simulink model "sensor_MAG_model"  (R2025b)
settings: Solver=FixedStepDiscrete  StartTime=0.0  StopTime=20  FixedStep=0.001  RelTol=1e-3
undefined symbols (not defined in the file or in its folder): IMU_SAMPLE_RATE, MAG_RANGE, MAG_SAMPLE_RATE
settings Model: DataDictionary=SensorDict.sldd  Creator=89447  LastModifiedBy=89447
settings DataIOCC: ExternalInput=S  LoadExternalInput=on

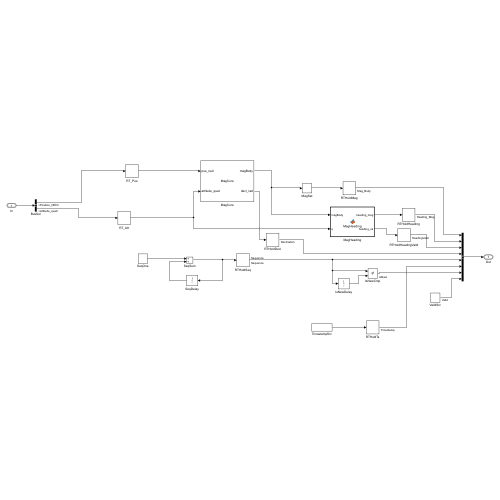
[thumbnail: Simulink's stored preview of the top-level diagram]
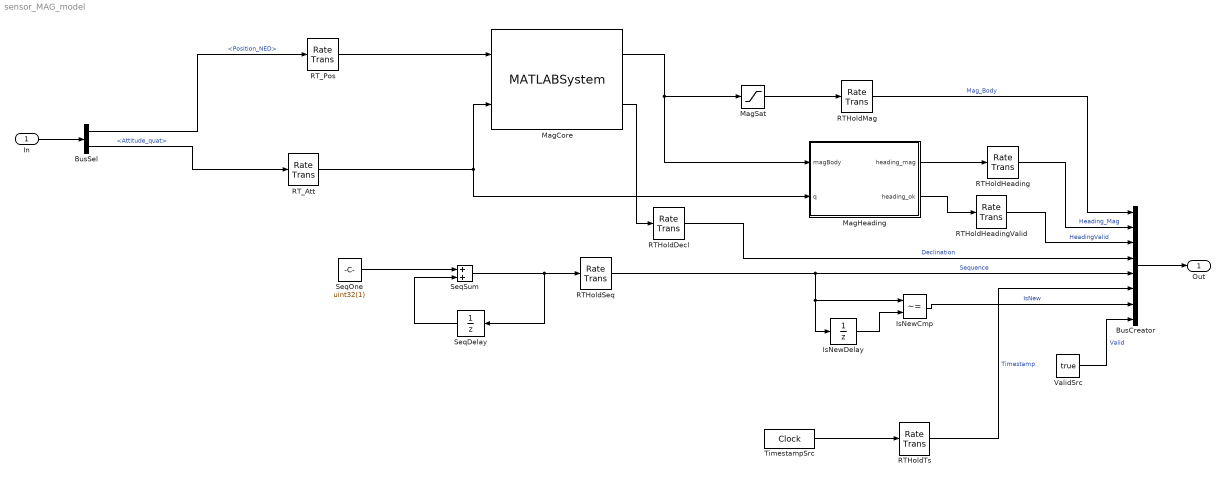
== system sensor_MAG_model ==
  In : Inport  OutDataTypeStr=Bus: DynamicModelBus
  BusCreator : BusCreator  Inputs=8  OutDataTypeStr=Bus: MagnetometerBus  NonVirtualBus=on
  BusSel : BusSelector  OutputSignals=Position_NED,Attitude_quat
  IsNewCmp : RelationalOperator  Operator=~=  OutDataTypeStr=boolean  RndMeth=Simplest  InputSameDT=off
  IsNewDelay : UnitDelay  SampleTime=1/double(IMU_SAMPLE_RATE)  HasFrameUpgradeWarning=on
  MagCore : MATLABSystem  System=MagCore  SampleRate=100  AxesMisalignment=100 * eye( 3 )  Seed=77101  RefLat=0  RefLon=10  WmmEpoch=2025  ConstantBias=[ 0, 0, 0 ]  NoiseDensity=[ 0, 0, 0 ]  BiasInstability=[ 0, 0, 0 ]  RandomWalk=[ 0, 0, 0 ]  TemperatureBias=[ 0, 0, 0 ]  TemperatureScaleFactor=[ 0, 0, 0 ]  Temperature=25  SimulateUsing=Interpreted execution
      mask Type: MagCore
  MagHeading : MATLAB Function  TreatAsAtomicUnit=on
  MagSat : Saturate  UpperLimit=MAG_RANGE  LowerLimit=-MAG_RANGE
  RTHoldDecl : RateTransition  OutPortSampleTime=1/double(IMU_SAMPLE_RATE)
  RTHoldHeading : RateTransition  OutPortSampleTime=1/double(IMU_SAMPLE_RATE)
  RTHoldHeadingValid : RateTransition  OutPortSampleTime=1/double(IMU_SAMPLE_RATE)
  RTHoldMag : RateTransition  OutPortSampleTime=1/double(IMU_SAMPLE_RATE)
  RTHoldSeq : RateTransition  OutPortSampleTime=1/double(IMU_SAMPLE_RATE)
  RTHoldTs : RateTransition  OutPortSampleTime=1/double(IMU_SAMPLE_RATE)
  RT_Att : RateTransition  OutPortSampleTime=1/double(MAG_SAMPLE_RATE)
  RT_Pos : RateTransition  OutPortSampleTime=1/double(MAG_SAMPLE_RATE)
  SeqDelay : UnitDelay  SampleTime=1/double(MAG_SAMPLE_RATE)  HasFrameUpgradeWarning=on
  SeqOne : Constant  Value=uint32(1)  OutDataTypeStr=uint32
  SeqSum : Sum
  TimestampSrc : DigitalClock  SampleTime=1/double(IMU_SAMPLE_RATE)
  ValidSrc : Constant  Value=true  OutDataTypeStr=boolean
  Out : Outport  OutDataTypeStr=Bus: MagnetometerBus
  wires:
  In/1 -> BusSel/1
  BusSel/1 -> RT_Pos/1  "<Position_NED>"
  BusSel/2 -> RT_Att/1  "<Attitude_quat>"
  RT_Pos/1 -> MagCore/1
  RT_Att/1 -> MagHeading/2(q), MagCore/2
  MagCore/1 -> MagHeading/1(magBody), MagSat/1
  MagSat/1 -> RTHoldMag/1
  MagHeading/1(heading_mag) -> RTHoldHeading/1
  MagHeading/2(heading_ok) -> RTHoldHeadingValid/1
  MagCore/2 -> RTHoldDecl/1
  SeqOne/1 -> SeqSum/1
  SeqDelay/1 -> SeqSum/2
  SeqSum/1 -> SeqDelay/1, RTHoldSeq/1
  RTHoldSeq/1 -> BusCreator/5, IsNewCmp/1, IsNewDelay/1  "Sequence"
  IsNewDelay/1 -> IsNewCmp/2
  TimestampSrc/1 -> RTHoldTs/1
  RTHoldMag/1 -> BusCreator/1  "Mag_Body"
  RTHoldHeading/1 -> BusCreator/2  "Heading_Mag"
  RTHoldHeadingValid/1 -> BusCreator/3  "HeadingValid"
  RTHoldDecl/1 -> BusCreator/4  "Declination"
  RTHoldTs/1 -> BusCreator/6  "Timestamp"
  IsNewCmp/1 -> BusCreator/7  "IsNew"
  ValidSrc/1 -> BusCreator/8  "Valid"
  BusCreator/1 -> Out/1

== matlab function sensor_MAG_model/MagHeading ==
  data: magBody input; heading_mag output; q input; heading_ok output
function [heading_mag, heading_ok] = MagHeading(magBody, q)
%#codegen
C_bn = quat2rotm(q(:).');
phi   = atan2(C_bn(3,2), C_bn(3,3));
theta = -asin(max(-1, min(1, C_bn(3,1))));
mx = magBody(1); my = magBody(2); mz = magBody(3);
num = -my*cos(phi) + mz*sin(phi);
den =  mx*cos(theta) + my*sin(phi)*sin(theta) + mz*cos(phi)*sin(theta);
heading_mag = atan2(num, den);
nrm = sqrt(mx*mx + my*my + mz*mz);
hor = sqrt(mx*mx + my*my);
heading_ok = (nrm > single(20)) && (nrm < single(80)) && (hor > single(5));
end
